simulink model "sf_temporal_logic_scheduler"  (R2025b)
settings: Solver=FixedStepDiscrete  StartTime=0.0  StopTime=5  RelTol=1e-3  EnableMultiTasking=on
model workspace (MAT data in the model file):
  deltat = 0.001
settings Model: Creator=The MathWorks, Inc.  LastModifiedBy=The MathWorks, Inc.
settings SolverCC: AlgebraicLoopSolver=TrustRegion  InsertRTBMode=Auto
settings DataIOCC: SaveFormat=Array  ReturnWorkspaceOutputs=off
settings OptimizationCC: ReuseModelBlockBuffer=off  ExpressionDepthLimit=2147483647.0  InitFltsAndDblsToZero=on  EfficientMapNaN2IntZero=off  LifeSpan=inf
settings DebuggingCC: SaveWithParameterizedLinksMsg=none  UnderspecifiedInitializationDetection=Classic  MergeDetectMultiDrivingBlocksExec=none  SignalResolutionControl=TryResolveAllWithWarning  SolverPrmCheckMsg=warning  InheritedTsInSrcMsg=none  MultiTaskDSMMsg=warning  MultiTaskCondExecSysMsg=none  FcnCallInpInsideContextMsg=warning  UnconnectedInputMsg=warning  UnconnectedOutputMsg=warning  UnconnectedLineMsg=warning  StateNameClashWarn=warning  SFUnexpectedBacktrackingDiag=warning  SFNoUnconditionalDefaultTransitionDiag=warning  SFExecutionAtInitializationDiag=none  ArithmeticOperatorsInVariantConditions=warning
settings HardwareCC: ProdBitPerPointer=32.0  ProdBitPerSizeT=32.0  ProdBitPerPtrDiffT=32.0  ProdLargestAtomicFloat=None  ProdIntDivRoundTo=Undefined  ProdEndianess=Unspecified  ProdWordSize=32.0  ProdHWDeviceType=32-bit Generic
settings ModelReferenceCC: EnableRefExpFcnMdlSchedulingChecks=on  PropagateSignalLabelsOutOfModel=off
settings SFSimCC: SFSimEcho=off  SimUseLocalCustomCode=off  SimParseCustomCode=off
settings RTWCC: RTWUseLocalCustomCode=off  GPUComputeCapability=3.5
settings CodeAppCC: StateflowObjectComments=on
settings GRTTargetCC: TargetFcnLib=ansi_tfl_tmw.mat  TargetLangStandard=C89/C90 (ANSI)  CombineOutputUpdateFcns=off  GRTInterface=on
settings ConfigComp: CovMetricSettings=dw  CovSaveCumulativeToWorkspaceVar=on  CovSaveSingleToWorkspaceVar=on  CovExternalEMLEnable=off  CovSFcnEnable=off

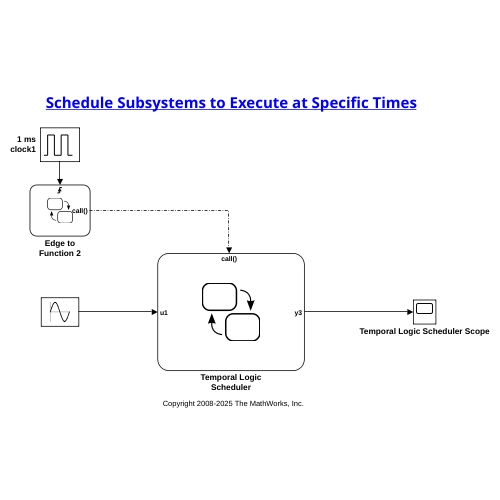
[thumbnail: Simulink's stored preview of the top-level diagram]
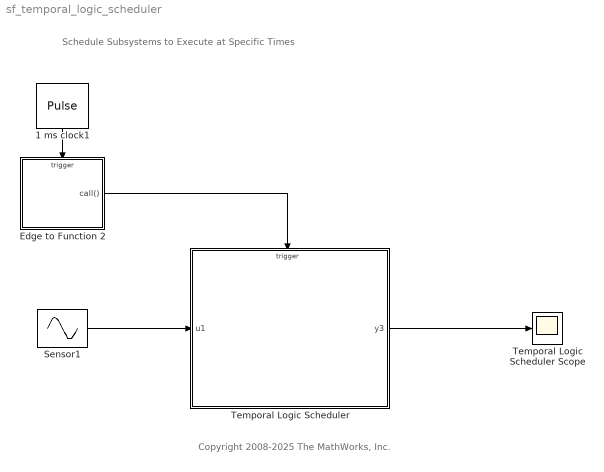
== system sf_temporal_logic_scheduler ==
  note: Copyright 2008-2025 The MathWorks, Inc.
  note: Schedule Subsystems to Execute at Specific Times
  1 ms clock1 : DiscretePulseGenerator  PulseType=Time based  Period=0.001  PulseWidth=10
  Edge to Function 2 : Stateflow chart  TreatAsAtomicUnit=on
  Sensor1 : Sin  Frequency=40  Phase=-pi/8
  Temporal Logic Scheduler : Stateflow chart  TreatAsAtomicUnit=on
  Temporal Logic Scheduler Scope : Scope
      settings: TimeSpan=0.7  ActiveDisplayYMinimum=-0.8  ActiveDisplayYMaximum=0.8  DataLoggingVariableName=ScopeData2
  wires:
  Temporal Logic Scheduler/1(y3) -> Temporal Logic Scheduler Scope/1
  Sensor1/1 -> Temporal Logic Scheduler/1(u1)
  Edge to Function 2/1(call()) -> Temporal Logic Scheduler/Trigger
  1 ms clock1/1 -> Edge to Function 2/Trigger

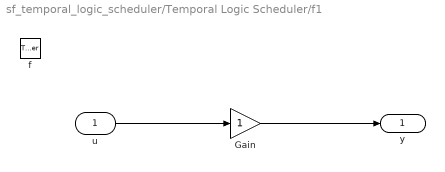
== system sf_temporal_logic_scheduler/Temporal Logic Scheduler/f1 ==
  u : Inport
  f : TriggerPort  TriggerType=function-call  VariantControl=(inherit)
      settings: CopyFcn=Stateflow.SLINSF.SimulinkMan.removeBlockPreDeleteFcn  PreDeleteFcn=Stateflow.SLINSF.SimulinkMan.unsafePredeleteFcn
  Gain : Gain
  y : Outport  VectorParamsAs1DForOutWhenUnconnected=off
  wires:
  u/1 -> Gain/1
  Gain/1 -> y/1

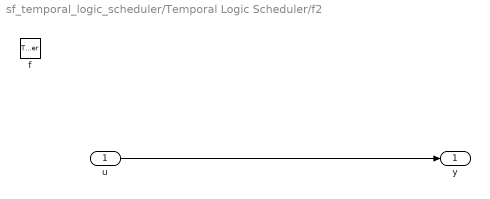
== system sf_temporal_logic_scheduler/Temporal Logic Scheduler/f2 ==
  u : Inport
  f : TriggerPort  TriggerType=function-call  VariantControl=(inherit)
      settings: CopyFcn=Stateflow.SLINSF.SimulinkMan.removeBlockPreDeleteFcn  PreDeleteFcn=Stateflow.SLINSF.SimulinkMan.unsafePredeleteFcn
  y : Outport  InitialOutput=0  VectorParamsAs1DForOutWhenUnconnected=off
  wires:
  u/1 -> y/1

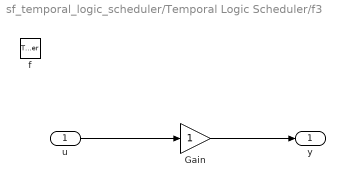
== system sf_temporal_logic_scheduler/Temporal Logic Scheduler/f3 ==
  u : Inport
  f : TriggerPort  TriggerType=function-call  VariantControl=(inherit)
      settings: CopyFcn=Stateflow.SLINSF.SimulinkMan.removeBlockPreDeleteFcn  PreDeleteFcn=Stateflow.SLINSF.SimulinkMan.unsafePredeleteFcn
  Gain : Gain
  y : Outport  VectorParamsAs1DForOutWhenUnconnected=off
  wires:
  u/1 -> Gain/1
  Gain/1 -> y/1

== stateflow chart sf_temporal_logic_scheduler/Edge to Function 2 ==
  settings: executeAtInitialization=1
  (default) -> (junction 2) : {call;}
  events: edge input RISING_EDGE_EVENT; call output FUNCTION_CALL_EVENT

== stateflow chart sf_temporal_logic_scheduler/Temporal Logic Scheduler ==
  settings: executeAtInitialization=1
  state y = f1(u) [function]
  state FastScheduler
    du: y = u1-y2;
    on every(1,call): y1 = f1(y) ;
    on every(2,call): y2 = f2(y1);
    on every(4,call): y3 = f3(y2);
  state y = f2(u) [function]
  state SlowScheduler
    du: y = u1-y2;
    on every(8,call): y1 = f1(y);
    on every(16,call): y2 = f2(y1);
    on every(32,call): y3 = f3(y2);
  state y = f3(u) [function]
  (default) -> FastScheduler
  SlowScheduler -> FastScheduler : after(100,call)
  FastScheduler -> SlowScheduler : after(100,call)
  data: u function_input; y function_output; u function_input; y function_output; u function_input; y function_output; y local double; u1 input; y1 local double; y2 local double; y3 output double
  events: call input FUNCTION_CALL_EVENT
